simulink model "dc_motor_discrete_pi_controller"  (R2024b)
settings: Solver=FixedStepAuto  StartTime=0.0  StopTime=10.0  FixedStep=0.01  RelTol=1e-3  EnableMultiTasking=on
undefined symbols (not defined in the file or in its folder): p
libraries: slpidlib x1
settings Model: Creator=Taha  LastModifiedBy=Taha
settings SolverCC: AutoInsertRateTranBlk=on
settings OptimizationCC: DefaultParameterBehavior=Inlined  UseDivisionForNetSlopeComputation=on  GainParamInheritBuiltInType=on  UseFloatMulNetSlope=on  InlineInvariantSignals=on  PassReuseOutputArgsAs=Individual arguments  ZeroExternalMemoryAtStartup=off  ZeroInternalMemoryAtStartup=off  NoFixptDivByZeroProtection=on  EfficientFloat2IntCast=on  LifeSpan=1  OptimizeBlockOrder=speed  DifferentSizesBufferReuse=on  EfficientTunableParamExpr=on
settings DebuggingCC: ParameterTunabilityLossMsg=error
settings HardwareCC: ProdLongLongMode=on
settings SFSimCC: MATLABDynamicMemAlloc=off
settings RTWCC: Description=Embedded Coder  SystemTargetFile=ert.tlc  TemplateMakefile=ert_default_tmf  TargetLang=C++
settings CodeAppCC: ForceParamTrailComments=on  IgnoreCustomStorageClasses=off  OperatorAnnotations=on  SimulinkDataObjDesc=on  SFDataObjDesc=on  CustomSymbolStrGlobalVar=rt$N$M  CustomSymbolStrType=$N$M  CustomSymbolStrFcn=$N$M$F  CustomSymbolStrMacro=$N$M  InsertBlockDesc=on
settings ERTTargetCC: TargetLangStandard=C++11 (ISO)  GenerateSampleERTMain=on  IncludeMdlTerminateFcn=off  CombineSignalStateStructs=on  CodeInterfacePackaging=C++ class  SupportComplex=off  SupportContinuousTime=on  RootIOFormat=Structure reference  ERTCustomFileTemplate=example_file_process.tlc  ERTFilePackagingFormat=CompactWithDataFile

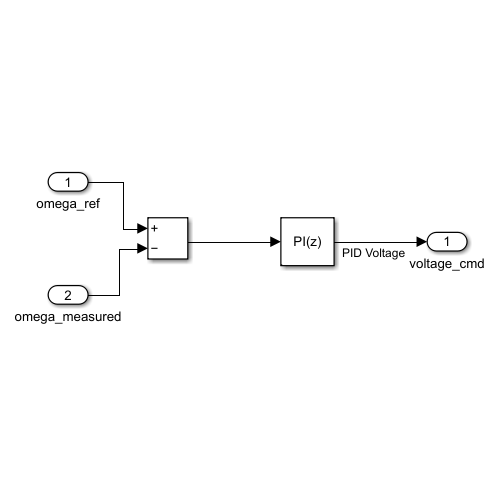
[thumbnail: Simulink's stored preview of the top-level diagram]
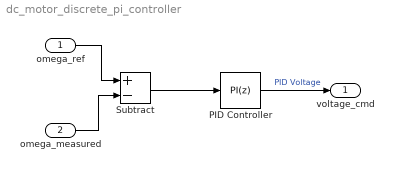
== system dc_motor_discrete_pi_controller ==
  omega_ref : Inport
  omega_measured : Inport  Port=2
  PID Controller : slpidlib/PID Controller  Controller=PI  Form=Parallel  TimeDomain=Discrete-time  UseExternalTs=off  SampleTime=0.01  IntegratorMethod=Forward Euler  FilterMethod=Forward Euler  ControllerParametersSource=internal  P=p.Kp  I=p.Ki  UseKiTs=off  D=0  UseExternalDerivativeSource=off  N=100  UseFilter=on  TunerSelectOption=Transfer Function Based (PID Tuner App)  InitialConditionSource=internal  InitialConditionForIntegrator=0  InitialConditionForFilter=0  DifferentiatorICPrevScaledInput=0  ExternalReset=none  TrackingMode=off  Kt=1  LimitOutput=off  SatLimitsSource=internal  UpperSaturationLimit=12  LowerSaturationLimit=0  LinearizeAsGain=on  AntiWindupMode=none  Kb=1  LimitIntegrator=off  UpperIntegratorSaturationLimit=inf  LowerIntegratorSaturationLimit=-inf  POutMin=[]  POutMax=[]  IOutMin=[]  IOutMax=[]  DOutMin=[]  DOutMax=[]  NOutMin=[]  NOutMax=[]  SumOutMin=[]  SumOutMax=[]  SaturationOutMin=[]  SaturationOutMax=[]  PParamMin=[]  PParamMax=[]  IParamMin=[]  IParamMax=[]  DParamMin=[]  DParamMax=[]  NParamMin=[]  NParamMax=[]  KbParamMin=[]  KbParamMax=[]  KtParamMin=[]  KtParamMax=[]  KbOutMin=[]  KbOutMax=[]  KtOutMin=[]  KtOutMax=[]  IntegratorOutMin=[]  IntegratorOutMax=[]  FilterOutMin=[]  FilterOutMax=[]  SumI1OutMin=[]  SumI1OutMax=[]  SumI2OutMin=[]  SumI2OutMax=[]  SumI3OutMin=[]  SumI3OutMax=[]  SumI4OutMin=[]  SumI4OutMax=[]  SumDOutMin=[]  SumDOutMax=[]  DifferentiatorOutMin=[]  DifferentiatorOutMax=[]  FilterDiffOutCoefMin=[]  FilterDiffOutCoefMax=[]  ReciprocalOutMin=[]  ReciprocalOutMax=[]  SumDenOutMin=[]  SumDenOutMax=[]  SumNumOutMin=[]  SumNumOutMax=[]  DivideOutMin=[]  DivideOutMax=[]  UdiffTsProdOutMin=[]  UdiffTsProdOutMax=[]  NTsProdOutMin=[]  NTsProdOutMax=[]  UintegralTsProdOutMin=[]  UintegralTsProdOutMax=[]  UngainTsProdOutMin=[]  UngainTsProdOutMax=[]  ClampingZeroOutDataTypeStr=Inherit: Inherit via back propagation  ClampingZeroOutMin=[]  ClampingZeroOutMax=[]  FilterDenConstantOutDataTypeStr=Inherit: Inherit via back propagation  FilterDenConstantOutMin=[]  FilterDenConstantOutMax=[]  PCopyOutDataTypeStr=Inherit: Inherit via back propagation  PCopyOutMin=[]  PCopyOutMax=[]  NCopyOutDataTypeStr=Inherit: Inherit via back propagation  NCopyOutMin=[]  NCopyOutMax=[]  IntegratorContinuousStateAttributes=''  IntegratorStateMustResolveToSignalObject=off  IntegratorRTWStateStorageClass=Auto  FilterContinuousStateAttributes=''  FilterStateMustResolveToSignalObject=off  FilterRTWStateStorageClass=Auto  ParallelPVariant=InternalParameters  IdealPVariant=Disabled  IVariant=InternalParameters  DVariant=Disabled  IntegratorVariant=Discrete  SatVariant=Disabled  AWVariant=Passthrough  PCopyVariant=Disabled  TRVariant=Disabled  FdbkBlocksVariant=Forward  IdealPFdbkVariant=Disabled  SatFdbkVariant=Disabled  DerivativeFilterVariant=Disabled  NVariant=Disabled  NCopyVariant=Disabled_SignalSpec  FilterICVariant=Disabled  IntegratorICVariant=InternalICs  ExternalResetVariant=Disabled  TRSumVariant=Passthrough  SumFdbkVariant=Disabled  SumVariant=Sum_PI  TsampFilterVariant=InternalTs  TsampNgainVariant=Passthrough  TsampIntegralVariant=Disabled_SignalSpec  ExternalSaturationOutDataTypeStr=Inherit: Same as second input  DerivativeSourceVariant=Disabled  PreIntVariant=InternalPreInt
  Subtract : Sum  Inputs=+-
  voltage_cmd : Outport
  wires:
  Subtract/1 -> PID Controller/1
  PID Controller/1 -> voltage_cmd/1  "PID Voltage"
  omega_ref/1 -> Subtract/1
  omega_measured/1 -> Subtract/2
